simulink model "motor_simulation"  (R2013b)
settings: Solver=ode45  StartTime=0.0  StopTime=Tsim_final  FixedStep=sim_step_size  RelTol=1e-3
values from neighbouring files (symbols this model uses):
  b = 0.01    [motor_parameters.m]    (also in motor_simulation_run.m = 0)
  J = 0.002    [motor_parameters.m]
  Kb = 0.7    [motor_parameters.m]
  Kt = 0.7    [motor_parameters.m]
  L = 0.004    [motor_parameters.m]
  R = 10    [motor_parameters.m]
  sim_step_size = TS    (= 0.015)    [motor_sim_impairments_run.m]    (also in motor_simulation_run.m = 0.0001)
  Tf = 0.02    [motor_parameters.m]    (also in motor_simulation_run.m = 0)
  Vsupply = 4.5    [motor_parameters.m]
settings Model: Creator=nding  LastModifiedBy=nding

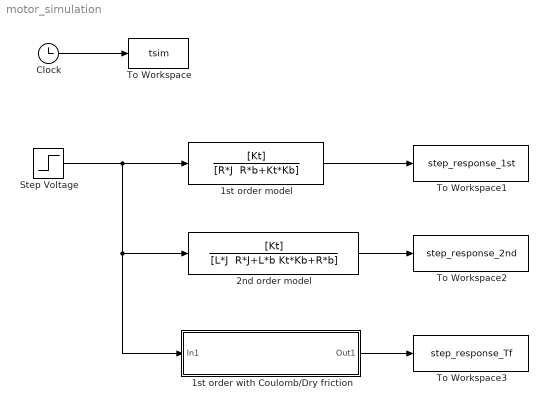
== system motor_simulation ==
  1st order model : TransferFcn  Numerator=[Kt]  Denominator="[R*J  R*b+Kt*Kb]"
  1st order with Coulomb/Dry friction : Subsystem  TreatAsAtomicUnit=on
  2nd order model : TransferFcn  Numerator=[Kt]  Denominator="[L*J  R*J+L*b Kt*Kb+R*b]"
  Clock : Clock
  Step Voltage : Step  Time=0  After=Vsupply  SampleTime=0
  To Workspace : ToWorkspace  VariableName=tsim  SampleTime=sim_step_size
  To Workspace1 : ToWorkspace  VariableName=step_response_1st  SampleTime=sim_step_size
  To Workspace2 : ToWorkspace  VariableName=step_response_2nd  SampleTime=sim_step_size
  To Workspace3 : ToWorkspace  VariableName=step_response_Tf  SampleTime=sim_step_size
  wires:
  Clock/1 -> To Workspace/1
  Step Voltage/1 -> 1st order with Coulomb/Dry friction/1(In1), 2nd order model/1, 1st order model/1
  1st order model/1 -> To Workspace1/1
  2nd order model/1 -> To Workspace2/1
  1st order with Coulomb/Dry friction/1(Out1) -> To Workspace3/1

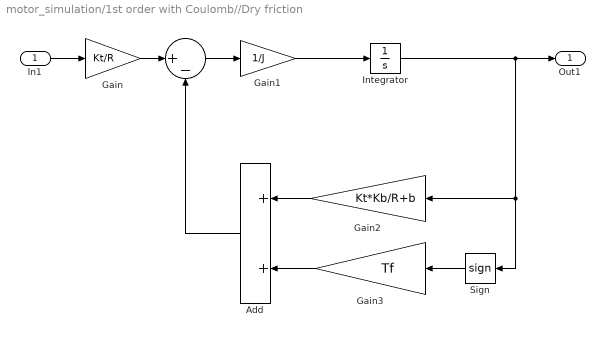
== system motor_simulation/1st order with Coulomb//Dry friction ==
  In1 : Inport
  " " : Sum  Inputs=|+-
  Add : Sum
  Gain : Gain  Gain=Kt/R
  Gain1 : Gain  Gain=1/J
  Gain2 : Gain  Gain=Kt*Kb/R+b
  Gain3 : Gain  Gain=Tf
  Integrator : Integrator
  Sign : Signum
  Out1 : Outport
  wires:
  In1/1 -> Gain/1
  Gain/1 -> " "/1
  " "/1 -> Gain1/1
  Gain1/1 -> Integrator/1
  Integrator/1 -> Sign/1, Gain2/1, Out1/1
  Add/1 -> " "/2
  Sign/1 -> Gain3/1
  Gain3/1 -> Add/2
  Gain2/1 -> Add/1
